simulink model "ssc_aircraft_elec"  (R2025a)
settings: Solver=ode23t  StartTime=0.0  StopTime=FlightProfileLength  RelTol=1e-3  AbsTol=1e-3  EnableMultiTasking=on
PreLoadFcn:
  | ssc_aircraft_elec_default_params
PostLoadFcn:
  | warning('off','physmod:common:gl:sli:rtp:InvalidNonValueReference');
  | warning off Simulink:Engine:SortDiscontinuityInAlgLoop
model workspace (MATLAB code in the model file):
  | v0                 = 0; % Initial vehicle speed
  | wheel_radius = 0.15; % Wheel radius
  | k                   = 1e-2; % Motor losses (W/(N*M)^2)
  | t_torque        = 0.02; % Electric motor time constant
  | rpm0             = 2000; % Engine initial speed demand
undefined symbols (not defined in the file): Based, Height, motor_ref_speed, PowerSystemChoice
libraries: fl_lib x34, nesl_utility x20, ee_lib x6, ssc_aircraft_elec_lib x2, batteryecm_lib x1, simulink x1
CloseFcn:
  | try,close(h1_ssc_aircraft_elec),end
  | clear h1_ssc_aircraft_elec
  | try,close(h2_ssc_aircraft_elec),end
  | clear h2_ssc_aircraft_elec
  | try,close(h3_ssc_aircraft_elec),end
  | clear h3_ssc_aircraft_elec
  | try,close(h4_ssc_aircraft_elec),end
  | clear h4_ssc_aircraft_elec
  | try,close(h5_ssc_aircraft_elec),end
  | clear h5_ssc_aircraft_elec
  | try,close(h6_ssc_aircraft_elec),end
  | clear h6_ssc_aircraft_elec
  | 
  | clear simlog_ssc_aircraft_elec
  | clear logsout_ssc_aircraft_elec
Description:
  | Electric Aircraft Component Sizing
  | 
  | Copyright 2017-2025 The MathWorks, Inc.
settings Model: FPTRunName=Active  Creator=MathWorks  LastModifiedBy=smiller
settings SolverCC: AutoScaleAbsTol=off  AlgebraicLoopSolver=TrustRegion
settings DataIOCC: InitialState=xBaseline  LimitDataPoints=on  MaxDataPoints=10000  SaveOperatingPoint=on  SaveFormat=Array  SignalLoggingSaveFormat=ModelDataLogs  ReturnWorkspaceOutputs=off  SignalLoggingName=logsout_ssc_aircraft_elec
settings OptimizationCC: ReuseModelBlockBuffer=off  ExpressionDepthLimit=2147483647.0  LifeSpan=inf
settings DebuggingCC: AlgebraicLoopMsg=none  UnderspecifiedInitializationDetection=Classic  MergeDetectMultiDrivingBlocksExec=none  FcnCallInpInsideContextMsg=warning  UnconnectedInputMsg=warning  UnconnectedOutputMsg=warning  UnconnectedLineMsg=warning  StateNameClashWarn=warning  PregeneratedLibrarySubsystemCodeDiagnostic=none  SFUnexpectedBacktrackingDiag=warning  SFNoUnconditionalDefaultTransitionDiag=warning  SFExecutionAtInitializationDiag=none  ArithmeticOperatorsInVariantConditions=warning
settings HardwareCC: ProdBitPerPointer=32.0  ProdBitPerSizeT=32.0  ProdBitPerPtrDiffT=32.0  ProdLargestAtomicFloat=None  ProdIntDivRoundTo=Undefined  ProdEndianess=Unspecified  ProdWordSize=32.0  ProdHWDeviceType=32-bit Generic
settings ModelReferenceCC: EnableRefExpFcnMdlSchedulingChecks=on  PropagateSignalLabelsOutOfModel=off
settings SFSimCC: SimUseLocalCustomCode=off  CustomCodeUndefinedFunction=UseInterfaceOnly
settings RTWCC: RTWUseLocalCustomCode=off  GPUComputeCapability=3.5  DLArmComputeVersion=19.05
settings CodeAppCC: StateflowObjectComments=on
settings GRTTargetCC: TargetLangStandard=C89/C90 (ANSI)  CombineOutputUpdateFcns=off  GRTInterface=on
settings ConfigComp: CovMetricSettings=dw  CovSaveCumulativeToWorkspaceVar=on  CovSaveSingleToWorkspaceVar=on  CovExternalEMLEnable=off
settings SimscapeCC: SimscapeNormalizeSystem=off  SimscapeLogType=all  SimscapeLogSimulationStatistics=on  SimscapeLogName=simlog_ssc_aircraft_elec  SimscapeLogDataHistory=10000.0

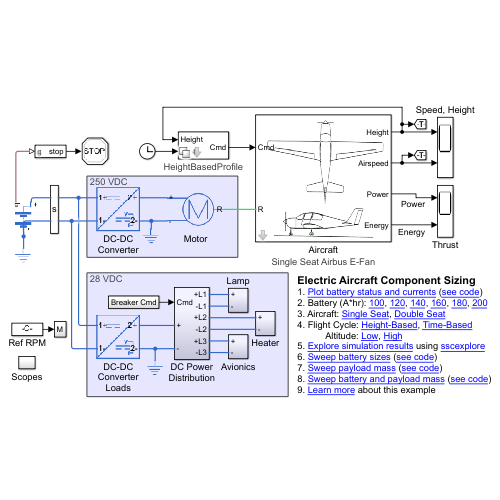
[thumbnail: Simulink's stored preview of the top-level diagram]
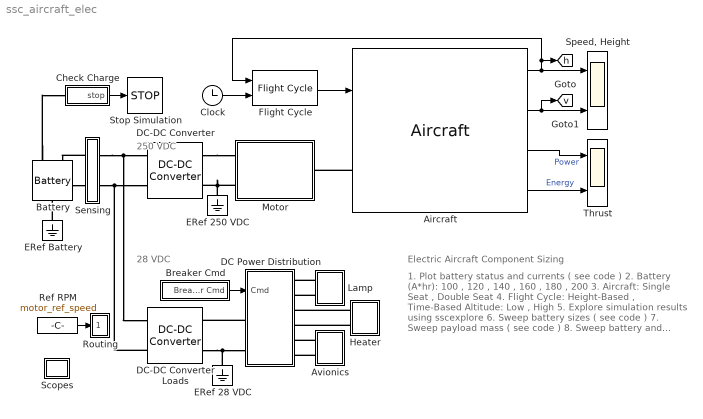
== system ssc_aircraft_elec ==
  note: 250 VDC
  note: 28 VDC
  note: Electric Aircraft Component Sizing
  note: 1. Plot battery status and currents ( see code )
      | 2. Battery (A*hr): 100 , 120 , 140 , 160 , 180 , 200
      | 3. Aircraft: Single Seat , Double Seat
      | 4. Flight Cycle: Height-Based , Time-Based
      | Altitude: Low , High
      | 5. Explore simulation results using sscexplore
      | 6. Sweep battery sizes ( see code )
      | 7. Sweep payload mass ( see code )
      | 8. Sweep battery and payload mass ( see code )
      | 9. Learn more about this example
  Aircraft : ssc_aircraft_elec_lib/Aircraft  Tag=PublishSubsystem  popup_aircraft_type=Single Seat Airbus E-Fan  aircraft_mass_cust=360  aircraft_wing_area_cust=10  aircraft_cl_cust=0.5  aircraft_cd_cust=0.05  battery_capacity=battery_capacity  battery_voltage=battery_vnom  battery_power_density=battery_pdensity  battery_mass=PowerSystemChoice.battery_capacity * PowerSystemChoice.battery_voltage / PowerSystemChoice.power_density  engine_system_mass=0  aircraft_max_thrust=max_thrust  aircraft_thrust_tau=thrust_tau  thrust_eff=thrust_eff  aircraft_h0=FlightProfileChoice.h0  aircraft_v0=0  earth_gravity=g_norm  checkbox_payload_mass=on  payload_mass=payload_mass
      settings: AttributesFormatString=%<popup_aircraft_type>
  Avionics : Subsystem
  Battery : batteryecm_lib/Battery  Vnom=201.6 V  prm_dir=1  R1_dis=2 Ohm  R1_ch=2 Ohm  R1=0.05 Ohm  prm_AH=2  AH=battery_capacity hr*A  V1=190 V  AH1=75 hr*A  prm_R2=1  R2=2000 Ohm  Tmeas=298.15 K  charge_measurement_port=simscape.enum.battery.enable.yes  prm_dyn=1  Rp1=0.005 Ohm  tau1=30 s  Rp2=0.005 Ohm  tau2=30 s  Rp3=0.005 Ohm  tau3=30 s  Rp4=0.005 Ohm  tau4=30 s  Rp5=0.005 Ohm  tau5=30 s  prm_fade=1  N_fade=100  AH_fade=45 hr*A  R1_fade=2.02 Ohm  R1_ch_fade=2.02 Ohm  V1_fade=10.35 V  prm_age=1  prm_age_OCV=1  OCV_age=0.9  SOC_age=60  Tmeas_age=298.15 K  delta_time_age_vec=[0] d  temperature_age_vec=[273] K  OCV_scaling_age=2.2134e6  OCV_offset_age=1.632e6  temp_exp_age=0.515833569 V  t_exp_age=0.75  Vnom_T2=12 V  R1_T2=2.2 Ohm  R1_T2_dis=2.2 Ohm  R1_T2_ch=2.2 Ohm  V1_T2=11.4 V  R2_T2=2200 Ohm  Rp1_T2=0.005 Ohm  tau1_T2=30 s  Rp2_T2=0.005 Ohm  tau2_T2=30 s  Rp3_T2=0.005 Ohm  tau3_T2=30 s  Rp4_T2=0.005 Ohm  tau4_T2=30 s  Rp5_T2=0.005 Ohm  tau5_T2=30 s  Tmeas2=273.15 K  thermal_port=simscape.enum.thermaleffects.omit  thermal_mass=30000 J/K  i_specify=off  i_priority=None  i=0 A  i_nominal_specify=off  i_nominal_value=1  i_nominal_unit=A  v_specify=off  v_priority=None  v=0 V  v_nominal_specify=off  v_nominal_value=1  v_nominal_unit=V  charge_specify=on  charge_priority=High  charge=battery_capacity hr*A  charge_nominal_specify=off  charge_nominal_value=1  charge_nominal_unit=A*hr  num_cycles_specify=off  num_cycles_priority=High  num_cycles=0  num_cycles_nominal_specify=off  num_cycles_nominal_value=1  num_cycles_nominal_unit=1  temperature_specify=off  temperature_priority=High  temperature=298.15 K  temperature_nominal_specify=off  temperature_nominal_value=1  temperature_nominal_unit=K
      settings: InternalSimscapePortConfiguration="{\"Bottom\":[],\"Left\":[{\"id\":\"p\",\"label\":\"+\",\"type\":\"foundation.electrical.electrical\"},{\"id\":\"q\",\"label\":\"q\",\"type\":\"output\"}],\"Right\":[{\"id\":\"n\",\"label\":\"-\",\"type\":\"foundation.electrical.electrical\"}],\"Top\":[]}"
  Breaker Cmd : Subsystem
  Check Charge : Subsystem  mask{q_battery_limit=20}
      mask prompts: q_battery_limit "Battery charge lower limit (A*hr)"
  Clock : Clock
  DC Power Distribution : Subsystem
  DC-DC Converter : ee_lib/Semiconductors & Converters/Converters/DC-DC Converter  Vref_option=ee.enum.converters.voltageref.internal  v_ref=250 V  P_rated=200 kW  droop_enabled=true  droop_param=ee.enum.converters.droop.value  droop=0.001 V/A  droop_percent=2  Vref_droop=10 V  reversible=ee.enum.converters.directionality.bidirectional  G_diode=1e-8 1/Ohm  P_fixed=100 W  losses_option=ee.enum.converters.lossesOption.proportionalToSquaredCurrent  eff_rated=97  tableOption=ee.enum.converters.lossTableOption.current  i_eff_vec=[1, 2, 3, 4] A  v_eff_vec=[15, 30, 45] V  eff_vec=[90, 80, 70, 60]  eff_2D_table=[90, 85, 80; 80, 75, 70; 70, 65, 60; 60, 55, 50]  model_dynamics=ee.enum.converters.dynamics.yes  tau=0.02 s  v_ini=250 V  v1_min=1 V  R1=1000 Ohm  R2=1000 Ohm  fault_condition=ee.enum.faults.faultInputCondition.greaterThan  fault_threshold=0.5  T_eff_vec=[280, 300, 320] K  eff_3D_table=repmat([66; 76; 80; 74], 1, 3, 3)  thermal_mass=100 J/K  initial_temperature=298.15 K
      settings: InternalSimscapePortConfiguration="{\"Bottom\":[],\"Left\":[{\"id\":\"p1\",\"label\":\"1+\",\"type\":\"foundation.electrical.electrical\"},{\"id\":\"n1\",\"label\":\"1-\",\"type\":\"foundation.electrical.electrical\"}],\"Right\":[{\"id\":\"p2\",\"label\":\"2+\",\"type\":\"foundation.electrical.electrical\"},{\"id\":\"n2\",\"label\":\"2-\",\"type\":\"foundation.electrical.electrical\"}],\"Top\":[]}"
  DC-DC Converter Loads : ee_lib/Semiconductors & Converters/Converters/DC-DC Converter  Vref_option=ee.enum.converters.voltageref.internal  v_ref=28 V  P_rated=4 kW  droop_enabled=true  droop_param=1  droop=0.01 V/A  droop_percent=2  Vref_droop=10 V  reversible=0  G_diode=1e-8 1/Ohm  P_fixed=100 W  losses_option=ee.enum.converters.lossesOption.proportionalToSquaredCurrent  eff_rated=80  tableOption=ee.enum.converters.lossTableOption.current  i_eff_vec=[1, 2, 3, 4] A  v_eff_vec=[15, 30, 45] V  eff_vec=[90, 80, 70, 60]  eff_2D_table=[90, 85, 80; 80, 75, 70; 70, 65, 60; 60, 55, 50]  model_dynamics=1  tau=0.02 s  v_ini=28 V  v1_min=1 V  R1=1000 Ohm  R2=1000 Ohm  fault_condition=1  fault_threshold=0.5  T_eff_vec=[280, 300, 320] K  eff_3D_table=repmat([66; 76; 80; 74], 1, 3, 3)  thermal_mass=100 J/K  initial_temperature=298.15 K
      settings: InternalSimscapePortConfiguration="{\"Bottom\":[],\"Left\":[{\"id\":\"p1\",\"label\":\"1+\",\"type\":\"foundation.electrical.electrical\"},{\"id\":\"n1\",\"label\":\"1-\",\"type\":\"foundation.electrical.electrical\"}],\"Right\":[{\"id\":\"p2\",\"label\":\"2+\",\"type\":\"foundation.electrical.electrical\"},{\"id\":\"n2\",\"label\":\"2-\",\"type\":\"foundation.electrical.electrical\"}],\"Top\":[]}"
  ERef 250 VDC : fl_lib/Electrical/Electrical Elements/Electrical Reference
  ERef 28 VDC : fl_lib/Electrical/Electrical Elements/Electrical Reference
  ERef Battery : fl_lib/Electrical/Electrical Elements/Electrical Reference
  Flight Cycle : ssc_aircraft_elec_lib/Flight Cycle  popup_flight_cycle_type=Height-Based  flight_cycle_max_height=FlightProfileChoice.FlightProfileHeight  flight_cycle_ascent_start_time=FlightProfileChoice.LevelFlightTime  flight_cycle_duration=FlightProfileChoice.FlightProfileLength  flight_cycle_ascent_duration=FlightProfileChoice.ClimbFlightTime
      settings: AttributesFormatString=%<ActiveVariant>
  Heater : Subsystem
  Lamp : Subsystem
  Motor : Subsystem  Tag=PublishSubsystem
      mask Display: image('Motor_IMAGE.png');
  Ref RPM : Constant  Value=motor_ref_speed
  Routing : Subsystem
  Scopes : Subsystem
  Sensing : Subsystem
      mask Display: disp('s');
  "Speed, Height" : Scope  NumInputPorts=2
      settings: ActiveDisplayYMinimum=-12.5  ActiveDisplayYMaximum=1112.5
  Stop Simulation : Stop
  Thrust : Scope  NumInputPorts=2
      settings: ActiveDisplayYMinimum=-2.69374  ActiveDisplayYMaximum=24.24364  DataLoggingMaxPoints=50000  DataLoggingVariableName=ScopeData6
  tag scope: h=global, v=global
  wires:
  Ref RPM/1 -> Routing/1(M)
  Aircraft/2 -> [v], "Speed, Height"/2
  Aircraft/1 -> Flight Cycle/1, [h], "Speed, Height"/1
  Aircraft/3 -> Thrust/1  "Power"
  Aircraft/4 -> Thrust/2  "Energy"
  Clock/1 -> Flight Cycle/2
  Flight Cycle/1 -> Aircraft/1
  Breaker Cmd/1(Breaker Cmd) -> DC Power Distribution/1(Cmd)
  Check Charge/1(stop) -> Stop Simulation/1
  connections:
  Aircraft/LConn1 -- Motor/LConn1
  DC-DC Converter/RConn1 -- Motor/RConn1
  DC Power Distribution/LConn1 -- DC-DC Converter Loads/RConn1
  Heater/LConn1 -- DC Power Distribution/RConn3
  Lamp/LConn2 -- DC Power Distribution/RConn2
  Lamp/LConn1 -- DC Power Distribution/RConn1
  Heater/LConn2 -- DC Power Distribution/RConn4
  DC-DC Converter Loads/RConn2 -- ERef 28 VDC/LConn1 -- DC Power Distribution/LConn2
  Motor/RConn2 -- ERef 250 VDC/LConn1 -- DC-DC Converter/RConn2
  Sensing/LConn1 -- Battery/LConn1
  Sensing/LConn2 -- Battery/RConn1 -- ERef Battery/LConn1
  Avionics/LConn1 -- DC Power Distribution/RConn5
  Avionics/LConn2 -- DC Power Distribution/RConn6
  Battery/LConn2 -- Check Charge/LConn1
  Sensing/RConn1 -- DC-DC Converter Loads/LConn1 -- DC-DC Converter/LConn1
  DC-DC Converter Loads/LConn2 -- Sensing/RConn2 -- DC-DC Converter/LConn2

== system ssc_aircraft_elec/Avionics ==
  Electrical Power : Subsystem
  Resistor : fl_lib/Electrical/Electrical Elements/Resistor  R=1.5 Ohm  i_specify=off  i_priority=None  i=0 A  i_nominal_specify=off  i_nominal_value=1  i_nominal_unit=A  v_specify=off  v_priority=None  v=0 V  v_nominal_specify=off  v_nominal_value=1  v_nominal_unit=V
  + : PMIOPort  Side=Left
  - : PMIOPort  Port=2  Side=Left
  connections:
  Electrical Power/LConn1 -- +/RConn1
  Resistor/LConn1 -- Electrical Power/RConn1
  Electrical Power/LConn2 -- Resistor/RConn1 -- -/RConn1

== system ssc_aircraft_elec/Breaker Cmd ==
  Avionics Breaker : Constant
  Heater Breaker OFF : Constant  Value=0
  Heater Breaker ON : Constant
  Lamp Breaker : Constant
  Mux1 : Mux  Inputs=3
  Switch : Switch  Threshold=800  SaturateOnIntegerOverflow=off  InputSameDT=off
  Breaker Cmd : Outport  VectorParamsAs1DForOutWhenUnconnected=off
  wires:
  Mux1/1 -> Breaker Cmd/1
  Avionics Breaker/1 -> Mux1/3
  Lamp Breaker/1 -> Mux1/1
  Switch/1 -> Mux1/2
  [h] -> Switch/2
  Heater Breaker ON/1 -> Switch/1
  Heater Breaker OFF/1 -> Switch/3

== system ssc_aircraft_elec/Check Charge ==
  Compare To Constant : simulink/Logic and Bit Operations/Compare To Constant  relop=<=  const=q_battery_limit  OutDataTypeStr=boolean
  PS-Simulink Converter : nesl_utility/PS-Simulink Converter  PhysicalDomain=network_engine_domain  SubClassName=ps_output  LeftPortType=input  RightPortType=output  PseudoPeriodic=off  Frequencies=[]  VectorFormat=1-D array  Unit=A*hr  AffineConversion=off
  q : PMIOPort  Side=Left
  stop : Outport  VectorParamsAs1DForOutWhenUnconnected=off
  tag scope: Chg_battery=global
  wires:
  PS-Simulink Converter/1 -> [Chg_battery], Compare To Constant/1
  Compare To Constant/1 -> stop/1
  connections:
  q/RConn1 -- PS-Simulink Converter/LConn1

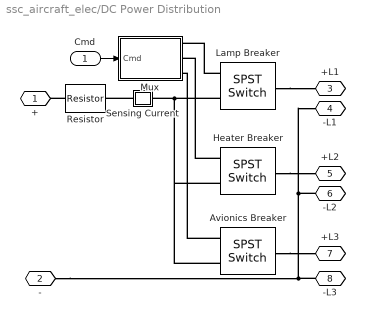
== system ssc_aircraft_elec/DC Power Distribution ==
  Cmd : Inport
  Avionics Breaker : ee_lib/Switches & Breakers/SPST Switch  R_closed=0.001 Ohm  G_open=1e-3 S  Threshold=0.5 V  Width=0 V  model_dynamics=0  t_on=1e-3 s  t_off=1e-3 s  initial_vT=0 V
      settings: InternalSimscapePortConfiguration="{\"Bottom\":[],\"Left\":[{\"id\":\"vT\",\"label\":\"vT\",\"type\":\"input\"},{\"id\":\"p\",\"label\":\"\",\"type\":\"foundation.electrical.electrical\"}],\"Right\":[{\"id\":\"n\",\"label\":\"\",\"type\":\"foundation.electrical.electrical\"}],\"Top\":[]}"
  Heater Breaker : ee_lib/Switches & Breakers/SPST Switch  R_closed=0.001 Ohm  G_open=1e-3 S  Threshold=0.5 V  Width=0 V  model_dynamics=0  t_on=1e-3 s  t_off=1e-3 s  initial_vT=0 V
      settings: InternalSimscapePortConfiguration="{\"Bottom\":[],\"Left\":[{\"id\":\"vT\",\"label\":\"vT\",\"type\":\"input\"},{\"id\":\"p\",\"label\":\"\",\"type\":\"foundation.electrical.electrical\"}],\"Right\":[{\"id\":\"n\",\"label\":\"\",\"type\":\"foundation.electrical.electrical\"}],\"Top\":[]}"
  Lamp Breaker : ee_lib/Switches & Breakers/SPST Switch  R_closed=0.001 Ohm  G_open=1e-3 S  Threshold=0.5 V  Width=0 V  model_dynamics=0  t_on=1e-3 s  t_off=1e-3 s  initial_vT=0 V
      settings: InternalSimscapePortConfiguration="{\"Bottom\":[],\"Left\":[{\"id\":\"vT\",\"label\":\"vT\",\"type\":\"input\"},{\"id\":\"p\",\"label\":\"\",\"type\":\"foundation.electrical.electrical\"}],\"Right\":[{\"id\":\"n\",\"label\":\"\",\"type\":\"foundation.electrical.electrical\"}],\"Top\":[]}"
  Mux : Subsystem
  Resistor : fl_lib/Electrical/Electrical Elements/Resistor  R=0.002 Ohm  i_specify=off  i_priority=None  i=0 A  i_nominal_specify=off  i_nominal_value=1  i_nominal_unit=A  v_specify=off  v_priority=None  v=0 V  v_nominal_specify=off  v_nominal_value=1  v_nominal_unit=V
  Sensing Current : Subsystem
      mask Display: disp('i')
  + : PMIOPort  Side=Left
  - : PMIOPort  Port=2  Side=Left
  +L1 : PMIOPort  Port=3  Side=Right
  -L1 : PMIOPort  Port=4  Side=Right
  +L2 : PMIOPort  Port=5  Side=Right
  -L2 : PMIOPort  Port=6  Side=Right
  +L3 : PMIOPort  Port=7  Side=Right
  -L3 : PMIOPort  Port=8  Side=Right
  wires:
  Cmd/1 -> Mux/1(Cmd)
  connections:
  Heater Breaker/LConn2 -- Avionics Breaker/LConn2 -- Sensing Current/RConn1 -- Lamp Breaker/LConn2
  -/RConn1 -- -L3/RConn1 -- -L2/RConn1 -- -L1/RConn1
  Lamp Breaker/RConn1 -- +L1/RConn1
  Heater Breaker/RConn1 -- +L2/RConn1
  Avionics Breaker/RConn1 -- +L3/RConn1
  Resistor/LConn1 -- +/RConn1
  Lamp Breaker/LConn1 -- Mux/RConn1
  Heater Breaker/LConn1 -- Mux/RConn2
  Avionics Breaker/LConn1 -- Mux/RConn3
  Sensing Current/LConn1 -- Resistor/RConn1

== system ssc_aircraft_elec/Heater ==
  Conductive Heat Transfer : fl_lib/Thermal/Thermal Elements/Conductive Heat Transfer  thermal_type=foundation.enum.ConstantVariableTabulated.Constant  wall_geometry=foundation.enum.ConductionWallGeometry.Planar  area=1e-4 m^2  thickness=0.1 m  d_in=0.05 m  d_out=0.1 m  L=1 m  th_cond_min=10 W/(K*m)  th_cond=401 W/(m*K)  th_cond_TLU=[413, 401, 392, 383, 371, 357, 342] W/(K*m)  temp_TLU=[200, 273, 400, 600, 800, 1000, 1200] K  T_specify=off  T_priority=None  T=0 K  T_nominal_specify=off  T_nominal_value=1  T_nominal_unit=K  Q_specify=off  Q_priority=None  Q=0 J/s  Q_nominal_specify=off  Q_nominal_value=1  Q_nominal_unit=J/s
  Convective Heat Transfer : fl_lib/Thermal/Thermal Elements/Convective Heat Transfer  thermal_type=foundation.enum.constant_variable.constant  area=1e-4 m^2  heat_tr_coeff=20 W/(m^2 * K)  min_heat_tr_coeff=1e-3 W/(K*m^2)  T_specify=off  T_priority=None  T=0 K  T_nominal_specify=off  T_nominal_value=1  T_nominal_unit=K  Q_specify=off  Q_priority=None  Q=0 J/s  Q_nominal_specify=off  Q_nominal_value=1  Q_nominal_unit=J/s
  Electrical Power : Subsystem
  Thermal Mass : fl_lib/Thermal/Thermal Elements/Thermal Mass  mass_type=foundation.enum.constant_variable.constant  mass=1 kg  sp_heat=447 J/kg/K  mass_min=1e-6 kg  num_ports=foundation.enum.numPorts2.one  m_specify=off  m_priority=High  m=1 kg  m_nominal_specify=off  m_nominal_value=1  m_nominal_unit=kg  T_specify=on  T_priority=High  T=300 K  T_nominal_specify=off  T_nominal_value=1  T_nominal_unit=K  Q_specify=off  Q_priority=None  Q=0 J/s  Q_nominal_specify=off  Q_nominal_value=1  Q_nominal_unit=J/s
  Thermal Reference : fl_lib/Thermal/Thermal Elements/Thermal Reference
  Thermal Resistor : fl_lib/Electrical/Electrical Elements/Thermal Resistor  R0=1 Ohm  T0=25 degC  alpha=5e-5 1/K  tc=10 s  K_d=1e-3 W/K  T_specify=on  T_priority=High  T=300 K  T_nominal_specify=off  T_nominal_value=1  T_nominal_unit=K
      settings: InternalSimscapePortConfiguration="{\"Bottom\":[],\"Left\":[{\"id\":\"H\",\"label\":\"H\",\"type\":\"foundation.thermal.thermal\"},{\"id\":\"p\",\"label\":\"+\",\"type\":\"foundation.electrical.electrical\"}],\"Right\":[{\"id\":\"n\",\"label\":\"-\",\"type\":\"foundation.electrical.electrical\"}],\"Top\":[]}"
  + : PMIOPort  Side=Left
  - : PMIOPort  Port=2  Side=Left
  connections:
  Electrical Power/RConn1 -- Thermal Resistor/LConn2
  Conductive Heat Transfer/RConn1 -- Convective Heat Transfer/LConn1 -- Thermal Mass/LConn1
  Thermal Resistor/LConn1 -- Conductive Heat Transfer/LConn1
  Convective Heat Transfer/RConn1 -- Thermal Reference/LConn1
  -/RConn1 -- Electrical Power/LConn2 -- Thermal Resistor/RConn1
  Electrical Power/LConn1 -- +/RConn1

== system ssc_aircraft_elec/Lamp ==
  Electrical Power : Subsystem
  Resistor : fl_lib/Electrical/Electrical Elements/Resistor  R=1 Ohm  i_specify=off  i_priority=None  i=0 A  i_nominal_specify=off  i_nominal_value=1  i_nominal_unit=A  v_specify=off  v_priority=None  v=0 V  v_nominal_specify=off  v_nominal_value=1  v_nominal_unit=V
  + : PMIOPort  Side=Left
  - : PMIOPort  Port=2  Side=Left
  connections:
  -/RConn1 -- Resistor/RConn1 -- Electrical Power/LConn2
  Resistor/LConn1 -- Electrical Power/RConn1
  Electrical Power/LConn1 -- +/RConn1

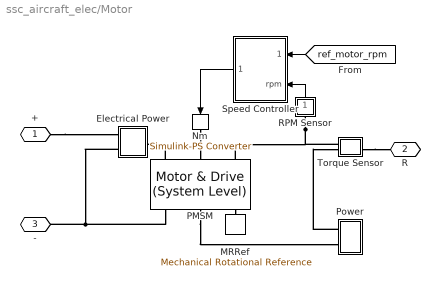
== system ssc_aircraft_elec/Motor ==
  Electrical Power : Subsystem
  MRRef : fl_lib/Mechanical/Rotational Elements/Mechanical Rotational Reference
  Nm : nesl_utility/Simulink-PS Converter  PhysicalDomain=network_engine_domain  SubClassName=ps_input  LeftPortType=input  RightPortType=output  PseudoPeriodic=off  Frequencies=[]  NoiseDistribution=none  NoiseParameters=[]  Unit=N*m  AffineConversion=off  FilteringAndDerivatives=zero  SimscapeFilterOrder=1  InputFilterTimeConstant=.001  UdotUserProvided=1
  PMSM : ee_lib/Electromechanical/Motor & Drive (System Level)  torque_speed_param=1  overtorque_param=ee.enum.electromech.overtorque.no  T_t=[ 0.9 0.8 0.7 0 ]*500 N*m  T_t_intermittent=[.36, .32, .28, 0] N*m  T_t_2D=[.09, .09, .09; .08, .08, .08; .07, .07, .07; 0, 0, 0] N*m  T_t_intermittent_2D=[.36, .36, .36; .32, .32, .32; .28, .28, .28; 0, 0, 0] N*m  w_t=[ 0 3.75e+3 7.5e+3 8e+3 ] rpm  vdc_t=[6, 12, 24] V  torque_max=0.1 N*m  power_max=30 W  torque_max_intermittent=0.4 N*m  power_max_intermittent=120 W  time_overtorque=30 s  time_recover=60 s  Tc=0.02 s  EnableSwitch=simscape.enum.onoff.off  losses_param=1  eff=95  w_eff=3.75e+3 rpm  T_eff=400 N*m  Piron=0 W  Pbase=0 W  w_eff_vec=[-8000 -4000 0 4000 8000] rpm  T_eff_vec=[0 0.03 0.06 0.09] N*m  v_eff_vec=[100, 250, 400] V  losses_mat=[1.49 1.67 2.21 3.10; 0.42 0.69 1.14 2.03; 0.06 0.24 0.78 1.68; 0.42 0.69 1.14 2.03; 1.49 1.67 2.21 3.10] W  efficiency_mat=[95 95 95 95; 95 95 95 95; 95 95 95 95; 95 95 95 95; 95 95 95 95]  losses_mat_3D=ones(5, 4, 3) W  efficiency_mat_3D=95 * ones(5, 4, 3)  Res=0 Ohm  J=0 kg*m^2  lam=1e-5 N*m/(rad/s)  speed0=2000 rpm  faulted_specify=off  faulted_priority=None  faulted=0  faulted_nominal_specify=off  faulted_nominal_value=1  faulted_nominal_unit=1  isSwitchedOff_specify=off  isSwitchedOff_priority=None  isSwitchedOff=0  isSwitchedOff_nominal_specify=off  isSwitchedOff_nominal_value=1  isSwitchedOff_nominal_unit=1  torqueLimitContinuous_specify=off  torqueLimitContinuous_priority=None  torqueLimitContinuous=0 N*m  torqueLimitContinuous_nominal_specify=off  torqueLimitContinuous_nominal_value=1  torqueLimitContinuous_nominal_unit=N*m  alpha=3.93e-3 1/K  Tmeas=25 degC  Tmeas2=125 degC  losses_mat_T2=[1.49, 1.74, 2.49, 3.74; .42, .67, 1.42, 2.67; .06, .31, 1.06, 2.31; .42, .67, 1.42, 2.67; 1.49, 1.74, 2.49, 3.74] W  efficiency_mat_T2=[95, 95, 95, 95; 95, 95, 95, 95; 95, 95, 95, 95; 95, 95, 95, 95; 95, 95, 95, 95]  losses_mat_3D_T2=ones(5, 4, 3) W  efficiency_mat_3D_T2=95 * ones(5, 4, 3)  thermal_mass=100 J/K  initial_temperature=25 degC
  Power : Subsystem
  RPM Sensor : Subsystem
      mask Display: disp('w')
  Speed Controller : Subsystem
  Torque Sensor : Subsystem
      mask Display: disp('trq');
  + : PMIOPort  Side=Right
  R : PMIOPort  Port=2  Side=Left
  - : PMIOPort  Port=3  Side=Right
  wires:
  Speed Controller/1(T_ref) -> Nm/1
  [ref_motor_rpm] -> Speed Controller/1(rpm_ref)
  RPM Sensor/1(rpm) -> Speed Controller/2(rpm)
  connections:
  PMSM/RConn2 -- Power/RConn2
  Nm/RConn1 -- PMSM/LConn2
  RPM Sensor/LConn1 -- Torque Sensor/LConn1 -- PMSM/LConn3
  Electrical Power/LConn2 -- -/RConn1 -- PMSM/RConn1
  PMSM/LConn1 -- Electrical Power/RConn1
  PMSM/RConn3 -- MRRef/LConn1
  +/RConn1 -- Electrical Power/LConn1
  Torque Sensor/RConn1 -- R/RConn1
  Power/RConn1 -- Torque Sensor/LConn2

== system ssc_aircraft_elec/Routing ==
  M : Inport
  Constant : Constant  Value=0
  tag scope: Fuel_Used=global, ref_motor_rpm=global
  wires:
  M/1 -> [ref_motor_rpm]
  Constant/1 -> [Fuel_Used]

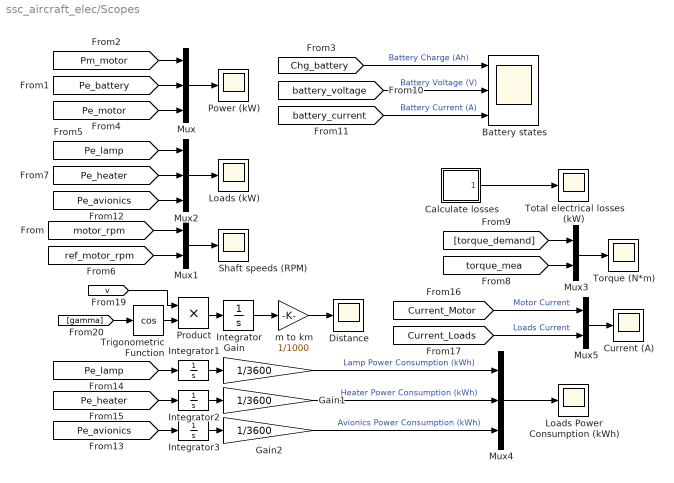
== system ssc_aircraft_elec/Scopes ==
  Battery states : Scope  NumInputPorts=3
      settings: ActiveDisplayYMinimum=10  ActiveDisplayYMaximum=110  DataLoggingVariableName=PureElecBatteryScopeData
  Calculate losses : Subsystem
  Current (A) : Scope
      settings: TimeSpan=20  ActiveDisplayYMinimum=-12.36171  ActiveDisplayYMaximum=111.25543  DataLoggingMaxPoints=50000  DataLoggingVariableName=PureElecCurrentData
  Distance : Scope
      settings: ActiveDisplayYMinimum=-9.67242  ActiveDisplayYMaximum=87.0518  DataLoggingVariableName=Distance  DataLoggingSaveFormat=Array
  Gain : Gain  Gain=1/3600
  Gain1 : Gain  Gain=1/3600
  Gain2 : Gain  Gain=1/3600
  Integrator{,1..3} (4 alike) : Integrator
  Loads (kW) : Scope
      settings: TimeSpan=20  ActiveDisplayYMinimum=-0.09663  ActiveDisplayYMaximum=0.86964  DataLoggingMaxPoints=50000
  Loads Power Consumption (kWh) : Scope
      settings: TimeSpan=20  ActiveDisplayYMinimum=-0.00246  ActiveDisplayYMaximum=0.00227  DataLoggingMaxPoints=50000  DataLoggingVariableName=PureElecLoadPowerConsumptionData
  Mux : Mux  Inputs=3
  Mux1 : Mux  Inputs=2
  Mux2 : Mux  Inputs=3
  Mux3 : Mux  Inputs=2
  Mux4 : Mux  Inputs=3
  Mux5 : Mux  Inputs=2
  Power (kW) : Scope
      settings: TimeSpan=20  ActiveDisplayYMinimum=-11.83354  ActiveDisplayYMaximum=106.49751  DataLoggingMaxPoints=50000  DataLoggingVariableName=ScopeData8
  Product : Product
  Shaft speeds (RPM) : Scope
      settings: ActiveDisplayYMinimum=1544.70029  ActiveDisplayYMaximum=2060.29139  DataLoggingMaxPoints=50000
  Torque (N*m) : Scope
      settings: TimeSpan=20  ActiveDisplayYMinimum=-49.6339  ActiveDisplayYMaximum=446.68415  DataLoggingMaxPoints=50000
  Total electrical losses (kW) : Scope
      settings: TimeSpan=20  ActiveDisplayYMinimum=-1.88992  ActiveDisplayYMaximum=29.92464  DataLoggingVariableName=ScopeData3
  Trigonometric Function : Trigonometry  Operator=cos
  m to km : Gain  Gain=1/1000
  wires:
  [Chg_battery] -> Battery states/1  "Battery Charge (Ah)"
  Calculate losses/1(Ploss) -> Total electrical losses (kW)/1
  [Pe_battery] -> Mux/2
  [motor_rpm] -> Mux1/1
  Mux1/1 -> Shaft speeds (RPM)/1
  Mux/1 -> Power (kW)/1
  Mux2/1 -> Loads (kW)/1
  [Pe_motor] -> Mux/3
  [Pm_motor] -> Mux/1
  [ref_motor_rpm] -> Mux1/2
  Mux3/1 -> Torque (N*m)/1
  [torque_demand] -> Mux3/1
  [torque_mea] -> Mux3/2
  [battery_voltage] -> Battery states/2  "Battery Voltage (V)"
  [battery_current] -> Battery states/3  "Battery Current (A)"
  [Pe_avionics] -> Mux2/3
  [Pe_lamp] -> Mux2/1
  [Pe_heater] -> Mux2/2
  [gamma] -> Trigonometric Function/1
  Trigonometric Function/1 -> Product/2
  Product/1 -> Integrator/1
  [v] -> Product/1
  Integrator/1 -> m to km/1
  m to km/1 -> Distance/1
  [Pe_lamp] -> Integrator1/1
  Mux4/1 -> Loads Power Consumption (kWh)/1
  [Pe_heater] -> Integrator2/1
  [Pe_avionics] -> Integrator3/1
  Integrator1/1 -> Gain/1
  Gain/1 -> Mux4/1  "Lamp Power Consumption (kWh)"
  Integrator2/1 -> Gain1/1
  Gain1/1 -> Mux4/2  "Heater Power Consumption (kWh)"
  Integrator3/1 -> Gain2/1
  Gain2/1 -> Mux4/3  "Avionics Power Consumption (kWh)"
  [Current_Motor] -> Mux5/1  "Motor Current"
  [Current_Loads] -> Mux5/2  "Loads Current"
  Mux5/1 -> Current (A)/1

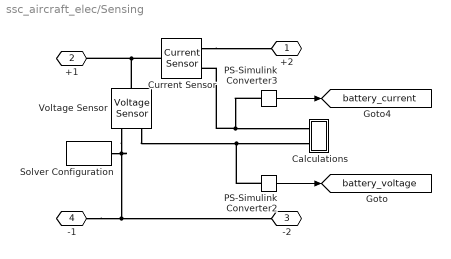
== system ssc_aircraft_elec/Sensing ==
  Calculations : Subsystem
  Current Sensor : fl_lib/Electrical/Electrical Sensors/Current Sensor
  PS-Simulink Converter2 : nesl_utility/PS-Simulink Converter  PhysicalDomain=network_engine_domain  SubClassName=ps_output  LeftPortType=input  RightPortType=output  PseudoPeriodic=off  Frequencies=[]  VectorFormat=1-D array  Unit=V  AffineConversion=off
  PS-Simulink Converter3 : nesl_utility/PS-Simulink Converter  PhysicalDomain=network_engine_domain  SubClassName=ps_output  LeftPortType=input  RightPortType=output  PseudoPeriodic=off  Frequencies=[]  VectorFormat=1-D array  Unit=A  AffineConversion=off
  Solver Configuration : nesl_utility/Solver Configuration  PhysicalDomain=network_engine_domain  SubClassName=solver  LeftPortType=input  RightPortType=generic  Tones=[]  Harmonics=[]  SimulateNoise=off  Profile=off  UseLocalSampling=off  EnableSwitchedLinearOptims=on  FrequencyDomain=off  UseCCode=off  RelTol=0.001  AbsTol=1e-06  MinStep=1e-09  ToWorkspace=off  RevertToSquareIcSolve=off  NumHomotopyIterations=100  PhasorMode=off  PhasorModeNumHarmonics=1  ConsistencySolver=NEWTON_FTOL  IndexReductionMethod=DerivativeReplacement  DoDC=off  ResidualTolerance=1e-9  ConsistencyTolSource=GLOBAL  ConsistencyAbsTol=0.001  ConsistencyRelTol=0.001  ConsistencyTolFactor=0.001  UseLocalSolver=off  LocalSolverChoice=NE_BACKWARD_EULER_ADVANCER  ResolveIndetEquations=on  FunctionEvalNumThread=1  LocalSolverSampleTime=0.01  DoFixedCost=off  MaxNonlinIter=3  MaxModeIter=2  ComputeImpulses=off  ImpulseIterations=2  LinearAlgebra=Sparse  LinearAlgebraNumThread=0  EquationFormulation=NE_TIME_EF  DelaysMemoryBudget=1024  AutomaticFiltering=on  FilteringTimeConstant=0.001  PartitionStorageMethod=AS_NEEDED  PartitionMemoryBudget=1024  PartitionMethod=FAST  MultibodyUseLocalSolver=off  MultibodyLocalSolverChoice=ODE1  MultibodyLocalSolverSampleTime=0.001
  Voltage Sensor : fl_lib/Electrical/Electrical Sensors/Voltage Sensor
  +2 : PMIOPort  Side=Right
  +1 : PMIOPort  Port=2  Side=Left
  -2 : PMIOPort  Port=3  Side=Right
  -1 : PMIOPort  Port=4  Side=Left
  tag scope: battery_current=global, battery_voltage=global
  wires:
  PS-Simulink Converter2/1 -> [battery_voltage]
  PS-Simulink Converter3/1 -> [battery_current]
  connections:
  Current Sensor/RConn2 -- +2/RConn1
  PS-Simulink Converter3/LConn1 -- Calculations/LConn1 -- Current Sensor/RConn1
  Voltage Sensor/RConn1 -- PS-Simulink Converter2/LConn1 -- Calculations/LConn2
  Current Sensor/LConn1 -- +1/RConn1 -- Voltage Sensor/LConn1
  Voltage Sensor/RConn2 -- Solver Configuration/RConn1 -- -1/RConn1 -- -2/RConn1

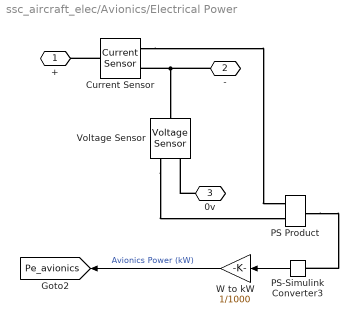
== system ssc_aircraft_elec/Avionics/Electrical Power ==
  " W to kW " : Gain  Gain=1/1000
  Current Sensor : fl_lib/Electrical/Electrical Sensors/Current Sensor
  PS Product : fl_lib/Physical Signals/Functions/PS Product
  PS-Simulink Converter3 : nesl_utility/PS-Simulink Converter  PhysicalDomain=network_engine_domain  SubClassName=ps_output  LeftPortType=input  RightPortType=output  PseudoPeriodic=off  Frequencies=[]  VectorFormat=1-D array  Unit=W  AffineConversion=off
  Voltage Sensor : fl_lib/Electrical/Electrical Sensors/Voltage Sensor
  + : PMIOPort  Side=Left
  - : PMIOPort  Port=2  Side=Right
  0v : PMIOPort  Port=3  Side=Left
  tag scope: Pe_avionics=global
  wires:
  PS-Simulink Converter3/1 -> " W to kW "/1
  " W to kW "/1 -> [Pe_avionics]  "Avionics Power (kW)"
  connections:
  Current Sensor/RConn1 -- PS Product/LConn1
  -/RConn1 -- Current Sensor/RConn2 -- Voltage Sensor/LConn1
  Current Sensor/LConn1 -- +/RConn1
  0v/RConn1 -- Voltage Sensor/RConn2
  Voltage Sensor/RConn1 -- PS Product/LConn2
  PS Product/RConn1 -- PS-Simulink Converter3/LConn1

== system ssc_aircraft_elec/DC Power Distribution/Mux ==
  Cmd : Inport
  Demux : Demux  Outputs=3
  Simulink-PS Converter1 : nesl_utility/Simulink-PS Converter  PhysicalDomain=network_engine_domain  SubClassName=ps_input  LeftPortType=input  RightPortType=output  PseudoPeriodic=off  Frequencies=[]  NoiseDistribution=none  NoiseParameters=[]  Unit=1  AffineConversion=off  FilteringAndDerivatives=zero  SimscapeFilterOrder=1  InputFilterTimeConstant=0.001  UdotUserProvided=1
  Simulink-PS Converter5 : nesl_utility/Simulink-PS Converter  PhysicalDomain=network_engine_domain  SubClassName=ps_input  LeftPortType=input  RightPortType=output  PseudoPeriodic=off  Frequencies=[]  NoiseDistribution=none  NoiseParameters=[]  Unit=1  AffineConversion=off  FilteringAndDerivatives=zero  SimscapeFilterOrder=1  InputFilterTimeConstant=0.001  UdotUserProvided=1
  Simulink-PS Converter6 : nesl_utility/Simulink-PS Converter  PhysicalDomain=network_engine_domain  SubClassName=ps_input  LeftPortType=input  RightPortType=output  PseudoPeriodic=off  Frequencies=[]  NoiseDistribution=none  NoiseParameters=[]  Unit=1  AffineConversion=off  FilteringAndDerivatives=zero  SimscapeFilterOrder=1  InputFilterTimeConstant=0.001  UdotUserProvided=1
  Lamp : PMIOPort  Side=Right
  Heat : PMIOPort  Port=2  Side=Right
  Avioincs : PMIOPort  Port=3  Side=Right
  wires:
  Demux/1 -> Simulink-PS Converter6/1
  Demux/2 -> Simulink-PS Converter5/1
  Demux/3 -> Simulink-PS Converter1/1
  Cmd/1 -> Demux/1
  connections:
  Simulink-PS Converter5/RConn1 -- Heat/RConn1
  Simulink-PS Converter6/RConn1 -- Lamp/RConn1
  Simulink-PS Converter1/RConn1 -- Avioincs/RConn1

== system ssc_aircraft_elec/DC Power Distribution/Sensing Current ==
  Current Sensor : fl_lib/Electrical/Electrical Sensors/Current Sensor
  PS-Simulink Converter1 : nesl_utility/PS-Simulink Converter  PhysicalDomain=network_engine_domain  SubClassName=ps_output  LeftPortType=input  RightPortType=output  PseudoPeriodic=off  Frequencies=[]  VectorFormat=1-D array  Unit=1  AffineConversion=off
  + : PMIOPort  Side=Left
  - : PMIOPort  Port=2  Side=Right
  tag scope: Current_Loads=global
  wires:
  PS-Simulink Converter1/1 -> [Current_Loads]
  connections:
  Current Sensor/RConn2 -- -/RConn1
  Current Sensor/LConn1 -- +/RConn1
  Current Sensor/RConn1 -- PS-Simulink Converter1/LConn1

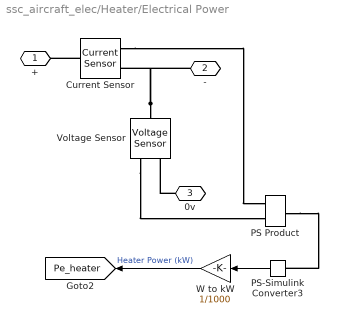
== system ssc_aircraft_elec/Heater/Electrical Power ==
  " W to kW " : Gain  Gain=1/1000
  Current Sensor : fl_lib/Electrical/Electrical Sensors/Current Sensor
  PS Product : fl_lib/Physical Signals/Functions/PS Product
  PS-Simulink Converter3 : nesl_utility/PS-Simulink Converter  PhysicalDomain=network_engine_domain  SubClassName=ps_output  LeftPortType=input  RightPortType=output  PseudoPeriodic=off  Frequencies=[]  VectorFormat=1-D array  Unit=W  AffineConversion=off
  Voltage Sensor : fl_lib/Electrical/Electrical Sensors/Voltage Sensor
  + : PMIOPort  Side=Left
  - : PMIOPort  Port=2  Side=Right
  0v : PMIOPort  Port=3  Side=Left
  tag scope: Pe_heater=global
  wires:
  " W to kW "/1 -> [Pe_heater]  "Heater Power (kW)"
  PS-Simulink Converter3/1 -> " W to kW "/1
  connections:
  PS Product/RConn1 -- PS-Simulink Converter3/LConn1
  Voltage Sensor/RConn1 -- PS Product/LConn2
  0v/RConn1 -- Voltage Sensor/RConn2
  Current Sensor/LConn1 -- +/RConn1
  Voltage Sensor/LConn1 -- Current Sensor/RConn2 -- -/RConn1
  Current Sensor/RConn1 -- PS Product/LConn1

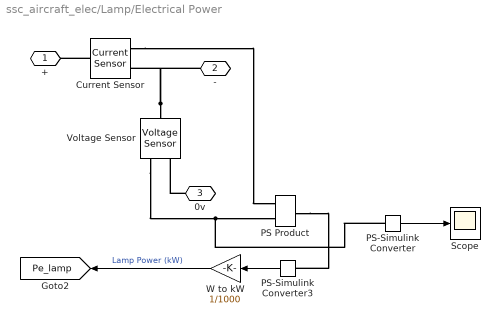
== system ssc_aircraft_elec/Lamp/Electrical Power ==
  " W to kW " : Gain  Gain=1/1000
  Current Sensor : fl_lib/Electrical/Electrical Sensors/Current Sensor
  PS Product : fl_lib/Physical Signals/Functions/PS Product
  PS-Simulink Converter : nesl_utility/PS-Simulink Converter  PhysicalDomain=network_engine_domain  SubClassName=ps_output  LeftPortType=input  RightPortType=output  PseudoPeriodic=off  Frequencies=[]  VectorFormat=1-D array  Unit=1  AffineConversion=off
  PS-Simulink Converter3 : nesl_utility/PS-Simulink Converter  PhysicalDomain=network_engine_domain  SubClassName=ps_output  LeftPortType=input  RightPortType=output  PseudoPeriodic=off  Frequencies=[]  VectorFormat=1-D array  Unit=W  AffineConversion=off
  Scope : Scope
      settings: ActiveDisplayYMinimum=27.04236  ActiveDisplayYMaximum=27.91869
  Voltage Sensor : fl_lib/Electrical/Electrical Sensors/Voltage Sensor
  + : PMIOPort  Side=Left
  - : PMIOPort  Port=2  Side=Right
  0v : PMIOPort  Port=3  Side=Left
  tag scope: Pe_lamp=global
  wires:
  " W to kW "/1 -> [Pe_lamp]  "Lamp Power (kW)"
  PS-Simulink Converter3/1 -> " W to kW "/1
  PS-Simulink Converter/1 -> Scope/1
  connections:
  PS Product/RConn1 -- PS-Simulink Converter3/LConn1
  Voltage Sensor/RConn1 -- PS-Simulink Converter/LConn1 -- PS Product/LConn2
  0v/RConn1 -- Voltage Sensor/RConn2
  Current Sensor/LConn1 -- +/RConn1
  Voltage Sensor/LConn1 -- Current Sensor/RConn2 -- -/RConn1
  Current Sensor/RConn1 -- PS Product/LConn1

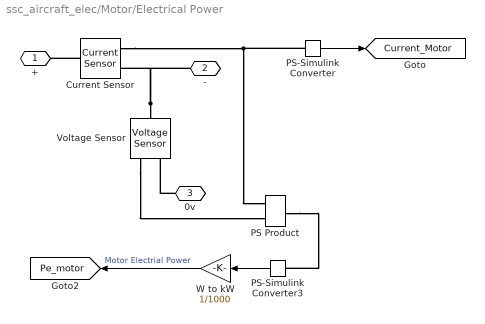
== system ssc_aircraft_elec/Motor/Electrical Power ==
  " W to kW " : Gain  Gain=1/1000
  Current Sensor : fl_lib/Electrical/Electrical Sensors/Current Sensor
  PS Product : fl_lib/Physical Signals/Functions/PS Product
  PS-Simulink Converter : nesl_utility/PS-Simulink Converter  PhysicalDomain=network_engine_domain  SubClassName=ps_output  LeftPortType=input  RightPortType=output  PseudoPeriodic=off  Frequencies=[]  VectorFormat=1-D array  Unit=1  AffineConversion=off
  PS-Simulink Converter3 : nesl_utility/PS-Simulink Converter  PhysicalDomain=network_engine_domain  SubClassName=ps_output  LeftPortType=input  RightPortType=output  PseudoPeriodic=off  Frequencies=[]  VectorFormat=1-D array  Unit=W  AffineConversion=off
  Voltage Sensor : fl_lib/Electrical/Electrical Sensors/Voltage Sensor
  + : PMIOPort  Side=Left
  - : PMIOPort  Port=2  Side=Right
  0v : PMIOPort  Port=3  Side=Left
  tag scope: Current_Motor=global, Pe_motor=global
  wires:
  " W to kW "/1 -> [Pe_motor]  "Motor Electrial Power"
  PS-Simulink Converter3/1 -> " W to kW "/1
  PS-Simulink Converter/1 -> [Current_Motor]
  connections:
  PS Product/RConn1 -- PS-Simulink Converter3/LConn1
  Voltage Sensor/RConn1 -- PS Product/LConn2
  0v/RConn1 -- Voltage Sensor/RConn2
  Current Sensor/LConn1 -- +/RConn1
  Voltage Sensor/LConn1 -- Current Sensor/RConn2 -- -/RConn1
  Current Sensor/RConn1 -- PS-Simulink Converter/LConn1 -- PS Product/LConn1

== system ssc_aircraft_elec/Motor/Power ==
  " W to kW " : Gain  Gain=1/1000
  PS Product : fl_lib/Physical Signals/Functions/PS Product
  PS-Simulink Converter3 : nesl_utility/PS-Simulink Converter  PhysicalDomain=network_engine_domain  SubClassName=ps_output  LeftPortType=input  RightPortType=output  PseudoPeriodic=off  Frequencies=[]  VectorFormat=1-D array  Unit=W  AffineConversion=off
  trq : PMIOPort  Side=Right
  w : PMIOPort  Port=2  Side=Right
  tag scope: Pm_motor=global
  wires:
  " W to kW "/1 -> [Pm_motor]  "Motor Mechanical Power"
  PS-Simulink Converter3/1 -> " W to kW "/1
  connections:
  PS Product/LConn1 -- trq/RConn1
  PS Product/LConn2 -- w/RConn1
  PS Product/RConn1 -- PS-Simulink Converter3/LConn1

== system ssc_aircraft_elec/Motor/RPM Sensor ==
  MRRef : fl_lib/Mechanical/Rotational Elements/Mechanical Rotational Reference
  Motion Sensor : fl_lib/Mechanical/Mechanical Sensors/Ideal Rotational Motion Sensor  reference=foundation.enum.MeasurementReference.difference  acceleration_port=false  velocity_port=true  position_port=true  wrap_angle=simscape.enum.onoff.off  offset=0 rad
  PS-Simulink Converter 2 : nesl_utility/PS-Simulink Converter  PhysicalDomain=network_engine_domain  SubClassName=ps_output  LeftPortType=input  RightPortType=output  PseudoPeriodic=off  Frequencies=[]  VectorFormat=1-D array  Unit=rpm  AffineConversion=off
  R : PMIOPort  Side=Left
  rpm : Outport  VectorParamsAs1DForOutWhenUnconnected=off
  tag scope: motor_rpm=global
  wires:
  PS-Simulink Converter 2/1 -> [motor_rpm], rpm/1
  connections:
  R/RConn1 -- Motion Sensor/LConn1
  Motion Sensor/RConn1 -- MRRef/LConn1
  Motion Sensor/RConn2 -- PS-Simulink Converter 2/LConn1

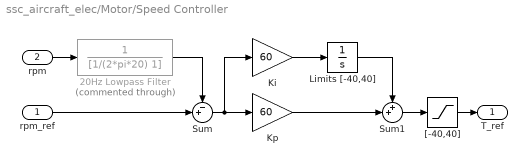
== system ssc_aircraft_elec/Motor/Speed Controller ==
  rpm_ref : Inport
  rpm : Inport  Port=2
  20Hz Lowpass Filter : TransferFcn  Commented=through  Denominator=[1/(2*pi*20) 1]
  Ki : Gain  Gain=60
  Kp : Gain  Gain=60
  Limits [-40,40] : Integrator  LimitOutput=on  UpperSaturationLimit=40  LowerSaturationLimit=-40
  Sum : Sum  Inputs=-+|
  Sum1 : Sum  Inputs=++|
  "[-40,40]" : Saturate  UpperLimit=400  LowerLimit=-400
  T_ref : Outport  VectorParamsAs1DForOutWhenUnconnected=off
  wires:
  "[-40,40]"/1 -> T_ref/1
  20Hz Lowpass Filter/1 -> Sum/1
  Limits [-40,40]/1 -> Sum1/1
  Kp/1 -> Sum1/2
  Ki/1 -> Limits [-40,40]/1
  Sum/1 -> Kp/1, Ki/1
  Sum1/1 -> "[-40,40]"/1
  rpm/1 -> 20Hz Lowpass Filter/1
  rpm_ref/1 -> Sum/2

== system ssc_aircraft_elec/Motor/Torque Sensor ==
  PS-Simulink Converter : nesl_utility/PS-Simulink Converter  PhysicalDomain=network_engine_domain  SubClassName=ps_output  LeftPortType=input  RightPortType=output  PseudoPeriodic=off  Frequencies=[]  VectorFormat=1-D array  Unit=1  AffineConversion=off
  Torque Sensor : fl_lib/Mechanical/Mechanical Sensors/Ideal Torque Sensor
  C : PMIOPort  Side=Right
  R : PMIOPort  Port=2  Side=Left
  trq : PMIOPort  Port=3  Side=Left
  tag scope: torque_mea=global
  wires:
  PS-Simulink Converter/1 -> [torque_mea]  "Measured Torque"
  connections:
  Torque Sensor/RConn2 -- trq/RConn1 -- PS-Simulink Converter/LConn1
  Torque Sensor/RConn1 -- C/RConn1
  Torque Sensor/LConn1 -- R/RConn1

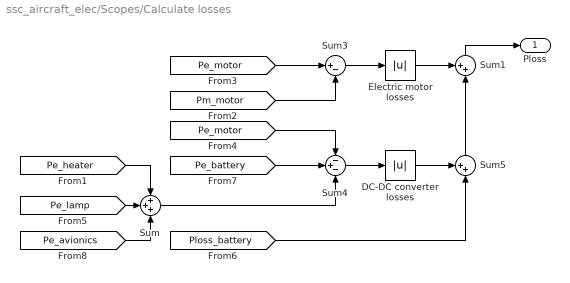
== system ssc_aircraft_elec/Scopes/Calculate losses ==
  " Electric motor losses" : Abs
  DC-DC converter losses : Abs
  Sum : Sum  Inputs=+++
  Sum1 : Sum  Inputs=++|
  Sum3 : Sum  Inputs=|+-
  Sum4 : Sum  Inputs=-+-
  Sum5 : Sum  Inputs=++|
  Ploss : Outport  VectorParamsAs1DForOutWhenUnconnected=off
  wires:
  [Ploss_battery] -> Sum5/2
  DC-DC converter losses/1 -> Sum5/1
  " Electric motor losses"/1 -> Sum1/1
  Sum/1 -> Sum4/3
  [Pe_motor] -> Sum4/1
  [Pe_battery] -> Sum4/2
  Sum5/1 -> Sum1/2
  Sum4/1 -> DC-DC converter losses/1
  Sum3/1 -> " Electric motor losses"/1
  [Pm_motor] -> Sum3/2
  [Pe_motor] -> Sum3/1
  Sum1/1 -> Ploss/1
  [Pe_heater] -> Sum/1
  [Pe_lamp] -> Sum/2
  [Pe_avionics] -> Sum/3

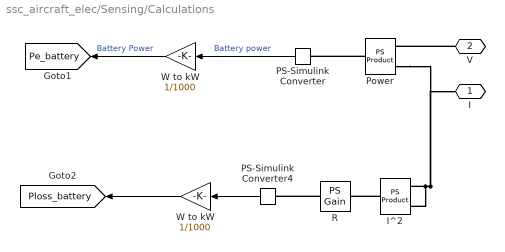
== system ssc_aircraft_elec/Sensing/Calculations ==
  " W to kW " : Gain  Gain=1/1000
  I^2 : fl_lib/Physical Signals/Functions/PS Product
  PS-Simulink Converter : nesl_utility/PS-Simulink Converter  PhysicalDomain=network_engine_domain  SubClassName=ps_output  LeftPortType=input  RightPortType=output  PseudoPeriodic=off  Frequencies=[]  VectorFormat=1-D array  Unit=W  AffineConversion=off
  PS-Simulink Converter4 : nesl_utility/PS-Simulink Converter  PhysicalDomain=network_engine_domain  SubClassName=ps_output  LeftPortType=input  RightPortType=output  PseudoPeriodic=off  Frequencies=[]  VectorFormat=1-D array  Unit=W  AffineConversion=off
  Power : fl_lib/Physical Signals/Functions/PS Product
  R : fl_lib/Physical Signals/Functions/PS Gain  gain=0.05 Ohm
  W to kW : Gain  Gain=1/1000
  I : PMIOPort  Side=Left
  V : PMIOPort  Port=2  Side=Left
  tag scope: Pe_battery=global, Ploss_battery=global
  wires:
  " W to kW "/1 -> [Ploss_battery]
  PS-Simulink Converter4/1 -> " W to kW "/1
  W to kW/1 -> [Pe_battery]  "Battery Power"
  PS-Simulink Converter/1 -> W to kW/1  "Battery power"
  connections:
  R/RConn1 -- PS-Simulink Converter4/LConn1
  I^2/RConn1 -- R/LConn1
  I^2/LConn1 -- I/RConn1 -- Power/LConn2 -- I^2/LConn2
  V/RConn1 -- Power/LConn1
  Power/RConn1 -- PS-Simulink Converter/LConn1
